simulink model "uz_sogipll"  (R2026b)
settings: Solver=FixedStepDiscrete  StopTime=5
settings Model: DataTypeOverride=Off  Creator=root  LastModifiedBy=root
settings DataIOCC: LimitDataPoints=on  SaveOutput=off  SaveTime=off
settings OptimizationCC: BlockReduction=off  ConditionallyExecuteInputs=off  DefaultParameterBehavior=Inlined  LifeSpan=inf
settings DebuggingCC: AlgebraicLoopMsg=error  AllowSymbolicDim=off  ArithmeticOperatorsInVariantConditions=warning  SFExecutionAtInitializationDiag=none  SFNoUnconditionalDefaultTransitionDiag=warning  SFUnexpectedBacktrackingDiag=warning  SingleTaskRateTransMsg=error  StrictBusMsg=ErrorOnBusTreatedAsVector
settings HardwareCC: ProdEndianess=Unspecified  ProdEqTarget=off  ProdHWDeviceType=ASIC/FPGA->ASIC/FPGA  ProdIntDivRoundTo=Undefined  ProdLargestAtomicFloat=None
settings SFSimCC: CustomCodeUndefinedFunction=UseInterfaceOnly  SimUseLocalCustomCode=off
settings RTWCC: RTWUseLocalCustomCode=off
settings CodeAppCC: StateflowObjectComments=on
settings GRTTargetCC: TargetLangStandard=C89/C90 (ANSI)
settings ConfigComp: CovExternalEMLEnable=off  CovSFcnEnable=off  CovSaveCumulativeToWorkspaceVar=on  CovSaveSingleToWorkspaceVar=on  CovScope=ReferencedModels

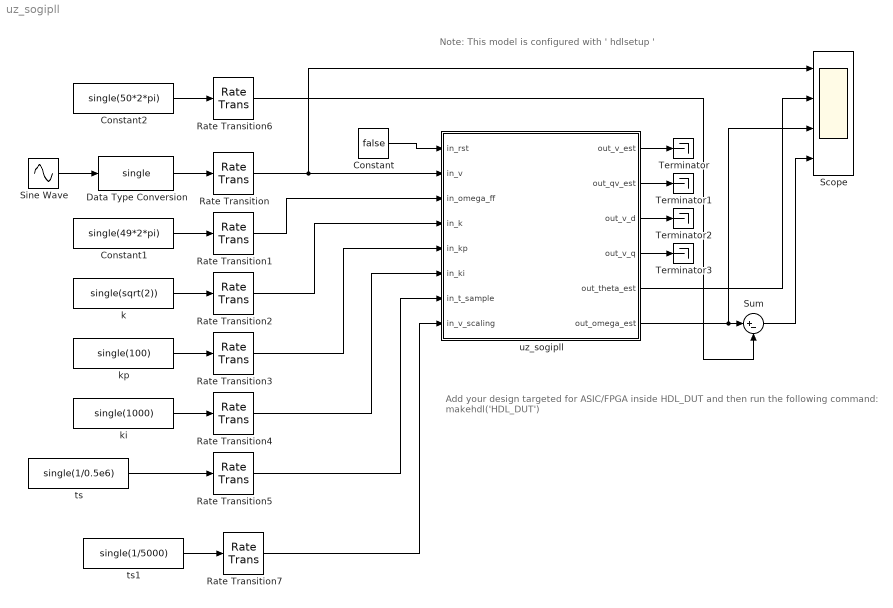
== system uz_sogipll ==
  note: Note: This model is configured with ' hdlsetup '
  note: Add your design targeted for ASIC/FPGA inside HDL_DUT and then run the following command:
      | makehdl('HDL_DUT')
  Constant : Constant  Value=false  OutDataTypeStr=boolean  SampleTime=-1
  Constant1 : Constant  Value=single(49*2*pi)
  Constant2 : Constant  Value=single(50*2*pi)
  Data Type Conversion : DataTypeConversion  OutDataTypeStr=single  SaturateOnIntegerOverflow=off  RndMeth=Floor
  Rate Transition : RateTransition  OutPortSampleTime=1/0.5e6
  Rate Transition{1..7} (7 alike) : RateTransition
  Scope : Scope  NumInputPorts=4
      settings: TimeSpan=10  ActiveDisplayYMinimum=-6250  ActiveDisplayYMaximum=6250  DataLoggingSaveFormat=Array
  Sine Wave : Sin  Amplitude=5000  Frequency=50*2*pi
  Sum : Sum  Inputs=|+-
  Terminator{,1..3} (4 alike) : Terminator
  k : Constant  Value=single(sqrt(2))
  ki : Constant  Value=single(1000)
  kp : Constant  Value=single(100)
  ts : Constant  Value=single(1/0.5e6)
  ts1 : Constant  Value=single(1/5000)
  uz_sogipll : Subsystem
  wires:
  Constant/1 -> uz_sogipll/1(in_rst)
  Sine Wave/1 -> Data Type Conversion/1
  Rate Transition/1 -> Scope/1, uz_sogipll/2(in_v)
  Constant1/1 -> Rate Transition1/1
  Rate Transition1/1 -> uz_sogipll/3(in_omega_ff)
  uz_sogipll/5(out_theta_est) -> Scope/2
  uz_sogipll/6(out_omega_est) -> Sum/1, Scope/3
  Rate Transition2/1 -> uz_sogipll/4(in_k)
  k/1 -> Rate Transition2/1
  kp/1 -> Rate Transition3/1
  ki/1 -> Rate Transition4/1
  Rate Transition3/1 -> uz_sogipll/5(in_kp)
  Rate Transition4/1 -> uz_sogipll/6(in_ki)
  Data Type Conversion/1 -> Rate Transition/1
  Sum/1 -> Scope/4
  ts/1 -> Rate Transition5/1
  Rate Transition5/1 -> uz_sogipll/7(in_t_sample)
  Constant2/1 -> Rate Transition6/1
  Rate Transition6/1 -> Sum/2
  ts1/1 -> Rate Transition7/1
  Rate Transition7/1 -> uz_sogipll/8(in_v_scaling)
  uz_sogipll/1(out_v_est) -> Terminator/1
  uz_sogipll/2(out_qv_est) -> Terminator1/1
  uz_sogipll/3(out_v_d) -> Terminator2/1
  uz_sogipll/4(out_v_q) -> Terminator3/1

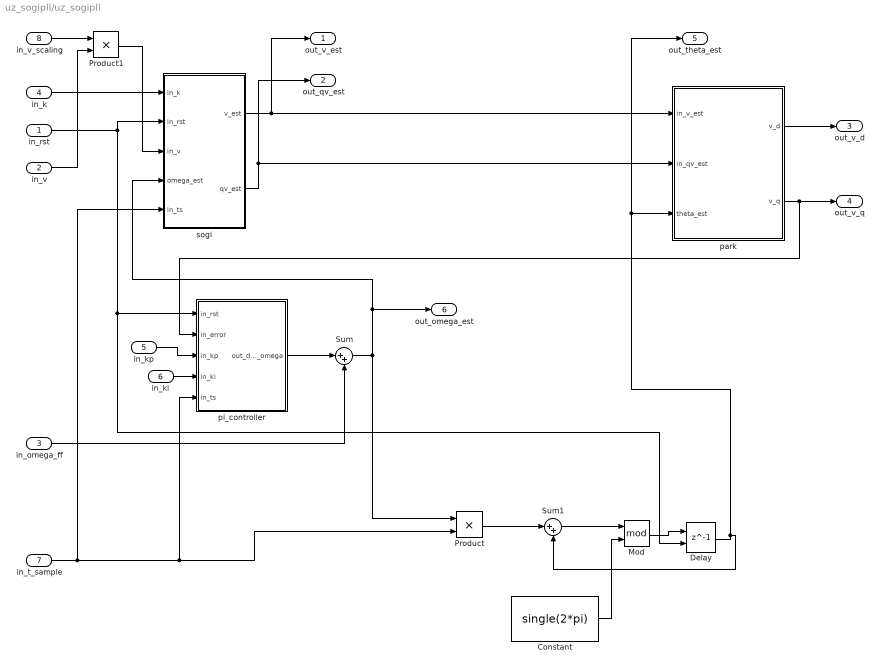
== system uz_sogipll/uz_sogipll ==
  in_rst : Inport
  in_v : Inport  Port=2
  in_omega_ff : Inport  Port=3
  in_k : Inport  Port=4
  in_kp : Inport  Port=5
  in_ki : Inport  Port=6
  in_t_sample : Inport  Port=7
  in_v_scaling : Inport  Port=8
  Constant : Constant  Value=single(2*pi)  SampleTime=-1
  Delay : Delay  DelayLength=1  ExternalReset=Level
      settings: InputPortMap=u0,r5
  Mod : Math  Operator=mod
  Product : Product
  Product1 : Product
  Sum : Sum  Inputs=|++
  Sum1 : Sum  Inputs=|++
  park : Subsystem
  pi_controller : Subsystem
  sogi : Subsystem
  out_v_est : Outport  VectorParamsAs1DForOutWhenUnconnected=off
  out_qv_est : Outport  Port=2  VectorParamsAs1DForOutWhenUnconnected=off
  out_v_d : Outport  Port=3  VectorParamsAs1DForOutWhenUnconnected=off
  out_v_q : Outport  Port=4  VectorParamsAs1DForOutWhenUnconnected=off
  out_theta_est : Outport  Port=5  VectorParamsAs1DForOutWhenUnconnected=off
  out_omega_est : Outport  Port=6  VectorParamsAs1DForOutWhenUnconnected=off
  wires:
  in_k/1 -> sogi/1(in_k)
  in_rst/1 -> Delay/2, pi_controller/1(in_rst), sogi/2(in_rst)
  sogi/1(v_est) -> park/1(in_v_est), out_v_est/1
  sogi/2(qv_est) -> park/2(in_qv_est), out_qv_est/1
  Delay/1 -> out_theta_est/1, park/3(theta_est), Sum1/2
  park/1(v_d) -> out_v_d/1
  park/2(v_q) -> pi_controller/2(in_error), out_v_q/1
  in_kp/1 -> pi_controller/3(in_kp)
  in_ki/1 -> pi_controller/4(in_ki)
  pi_controller/1(out_delta_omega) -> Sum/1
  in_omega_ff/1 -> Sum/2
  Sum/1 -> Product/1, sogi/4(omega_est), out_omega_est/1
  Product/1 -> Sum1/1
  Sum1/1 -> Mod/1
  Constant/1 -> Mod/2
  Mod/1 -> Delay/1
  in_t_sample/1 -> sogi/5(in_ts), pi_controller/5(in_ts), Product/2
  in_v_scaling/1 -> Product1/1
  in_v/1 -> Product1/2
  Product1/1 -> sogi/3(in_v)

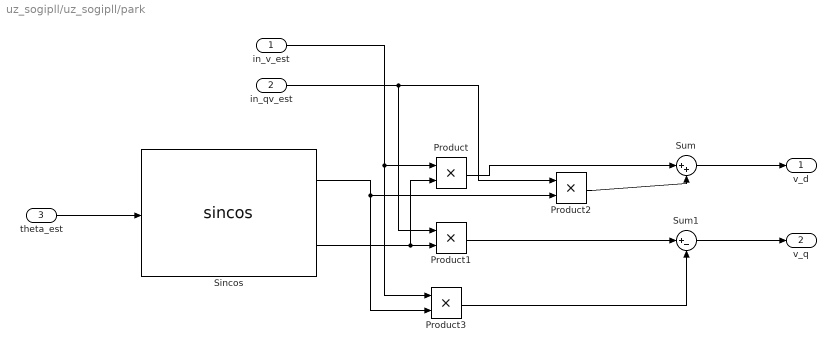
== system uz_sogipll/uz_sogipll/park ==
  in_v_est : Inport
  in_qv_est : Inport  Port=2
  theta_est : Inport  Port=3
  Product{,1..3} (4 alike) : Product
  Sincos : Trigonometry  Operator=sincos  OutputSignalType=real
  Sum : Sum  Inputs=|++
  Sum1 : Sum  Inputs=|+-
  v_d : Outport
  v_q : Outport  Port=2
  wires:
  Product1/1 -> Sum1/1
  Product2/1 -> Sum/2
  Product3/1 -> Sum1/2
  in_v_est/1 -> Product/1, Product3/1
  Sincos/1 -> Product2/2, Product3/2
  in_qv_est/1 -> Product2/1, Product1/1
  Sincos/2 -> Product/2, Product1/2
  Sum/1 -> v_d/1
  theta_est/1 -> Sincos/1
  Product/1 -> Sum/1
  Sum1/1 -> v_q/1

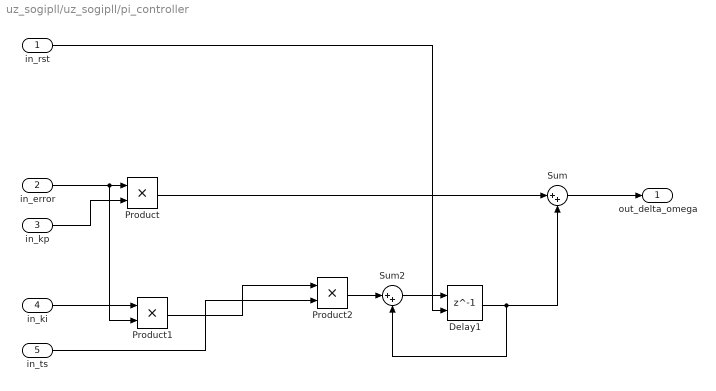
== system uz_sogipll/uz_sogipll/pi_controller ==
  in_rst : Inport
  in_error : Inport  Port=2
  in_kp : Inport  Port=3
  in_ki : Inport  Port=4
  in_ts : Inport  Port=5
  Delay1 : Delay  DelayLength=1  ExternalReset=Level
      settings: InputPortMap=u0,r5
  Product : Product
  Product1 : Product
  Product2 : Product
  Sum : Sum  Inputs=|++
  Sum2 : Sum  Inputs=|++
  out_delta_omega : Outport
  wires:
  in_error/1 -> Product1/2, Product/1
  in_kp/1 -> Product/2
  Product/1 -> Sum/1
  in_rst/1 -> Delay1/2
  in_ki/1 -> Product1/1
  Product1/1 -> Product2/1
  Delay1/1 -> Sum2/2, Sum/2
  Sum/1 -> out_delta_omega/1
  Product2/1 -> Sum2/1
  Sum2/1 -> Delay1/1
  in_ts/1 -> Product2/2

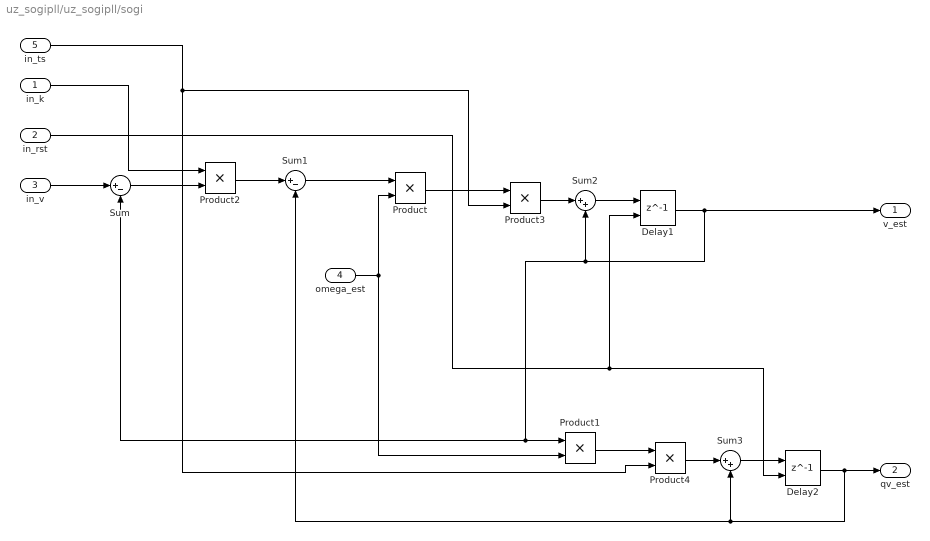
== system uz_sogipll/uz_sogipll/sogi ==
  in_k : Inport
  in_rst : Inport  Port=2
  in_v : Inport  Port=3
  omega_est : Inport  Port=4
  in_ts : Inport  Port=5
  Delay1 : Delay  DelayLength=1  ExternalReset=Level
      settings: InputPortMap=u0,r5
  Delay2 : Delay  DelayLength=1  ExternalReset=Level
      settings: InputPortMap=u0,r5
  Product{,1..4} (5 alike) : Product
  Sum : Sum  Inputs=|+-
  Sum1 : Sum  Inputs=|+-
  Sum2 : Sum  Inputs=|++
  Sum3 : Sum  Inputs=|++
  v_est : Outport
  qv_est : Outport  Port=2
  wires:
  in_k/1 -> Product2/1
  Product/1 -> Product3/1
  Sum/1 -> Product2/2
  Product2/1 -> Sum1/1
  omega_est/1 -> Product/2, Product1/2
  in_rst/1 -> Delay2/2, Delay1/2
  Delay1/1 -> Sum/2, Product1/1, Sum2/2, v_est/1
  Sum1/1 -> Product/1
  in_v/1 -> Sum/1
  Delay2/1 -> qv_est/1, Sum3/2, Sum1/2
  Product3/1 -> Sum2/1
  Sum2/1 -> Delay1/1
  in_ts/1 -> Product3/2, Product4/2
  Product4/1 -> Sum3/1
  Sum3/1 -> Delay2/1
  Product1/1 -> Product4/1
